simulink model "DiSiUp_1lab_1_1"  (R2025b)
settings: Solver=VariableStepAuto  StartTime=0.0  StopTime=5  RelTol=1e-8
undefined symbols (not defined in the file): K_fb
settings Model: Creator=waltanmari  LastModifiedBy=waltanmari

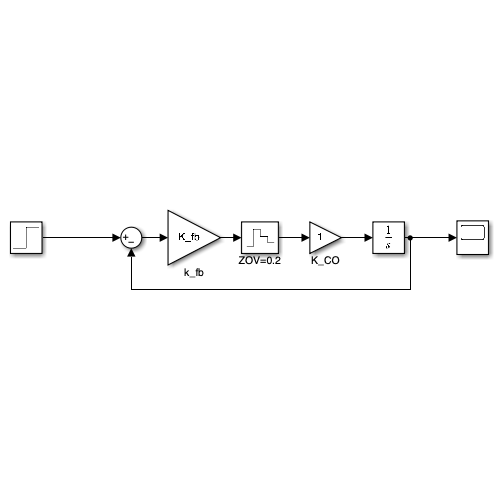
[thumbnail: Simulink's stored preview of the top-level diagram]
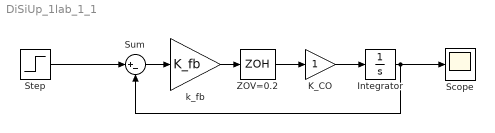
== system DiSiUp_1lab_1_1 ==
  Integrator : Integrator
  K_CO : Gain
  Scope : Scope
      settings: ActiveDisplayYMinimum=-0.1625  ActiveDisplayYMaximum=1.4625000000000004
  Step : Step  Time=0  SampleTime=0
  Sum : Sum  Inputs=|+-
  ZOV=0.2 : ZeroOrderHold  SampleTime=0.2
  k_fb : Gain  Gain=K_fb
  wires:
  Step/1 -> Sum/1
  Sum/1 -> k_fb/1
  Integrator/1 -> Sum/2, Scope/1
  K_CO/1 -> Integrator/1
  ZOV=0.2/1 -> K_CO/1
  k_fb/1 -> ZOV=0.2/1
